simulink model "Sistema3"  (R2026b)
settings: Solver=ode15s  StopTime=10  MaxStep=1E-2
libraries: slpidlib x1
settings Model: LastModifiedBy=Marcos Ancelmo
settings DataIOCC: DSMLogging=off  ReturnWorkspaceOutputs=off  SaveFormat=Array  SaveOutput=off  SignalLogging=off  TimeSaveName=t
settings DebuggingCC: AlgebraicLoopMsg=none  ArtificialAlgebraicLoopMsg=none  MaxConsecutiveZCsMsg=none

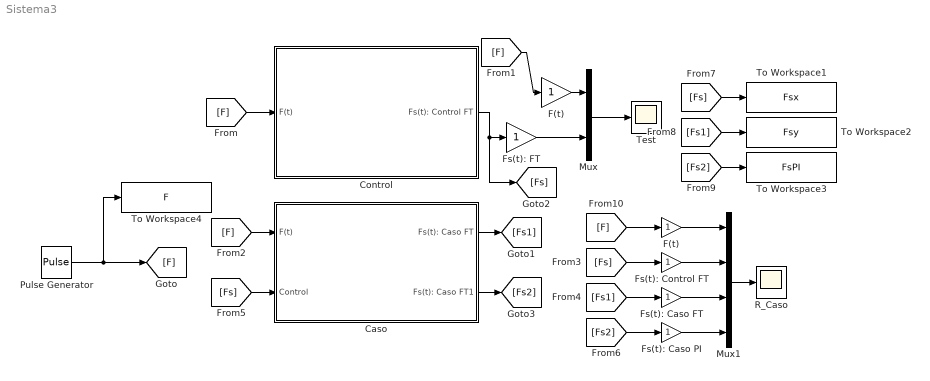
== system Sistema3 ==
  " F(t)" : Gain
  " Fs(t): Caso FT" : Gain
  " Fs(t): Caso PI" : Gain
  " Fs(t): Control FT" : Gain
  Caso : Subsystem
  Control : Subsystem
  F(t) : Gain
  Fs(t): FT : Gain
  Mux : Mux  Inputs=2
  Mux1 : Mux
  Pulse Generator : DiscretePulseGenerator  PulseType=Time based  Period=10  PulseWidth=10  PhaseDelay=1
  R_Caso : Scope
      settings: ActiveDisplayYMinimum=-0.12564340388071826  ActiveDisplayYMaximum=1.1250714893200797
  Test : Scope
      settings: ActiveDisplayYMinimum=-0.12500093230348591  ActiveDisplayYMaximum=1.1250001035892763
  To Workspace1 : ToWorkspace  VariableName=Fsx  SampleTime=-1
  To Workspace2 : ToWorkspace  VariableName=Fsy  SampleTime=-1
  To Workspace3 : ToWorkspace  VariableName=FsPI  SampleTime=-1
  To Workspace4 : ToWorkspace  VariableName=F  SampleTime=-1
  wires:
  Mux/1 -> Test/1
  [F] -> Control/1(F(t))
  Fs(t): FT/1 -> Mux/2
  Control/1(Fs(t): Control FT) -> [Fs], Fs(t): FT/1
  [F] -> Caso/1(F(t))
  Caso/1(Fs(t): Caso FT) -> [Fs1]
  Mux1/1 -> R_Caso/1
  [Fs] -> " Fs(t): Control FT"/1
  [Fs1] -> " Fs(t): Caso FT"/1
  Pulse Generator/1 -> To Workspace4/1, [F]
  [Fs] -> Caso/2(Control)
  Caso/2(Fs(t): Caso FT1) -> [Fs2]
  [Fs2] -> " Fs(t): Caso PI"/1
  [Fs] -> To Workspace1/1
  [Fs1] -> To Workspace2/1
  [Fs2] -> To Workspace3/1
  F(t)/1 -> Mux/1
  [F] -> F(t)/1
  [F] -> " F(t)"/1
  " Fs(t): Control FT"/1 -> Mux1/2
  " F(t)"/1 -> Mux1/1
  " Fs(t): Caso FT"/1 -> Mux1/3
  " Fs(t): Caso PI"/1 -> Mux1/4

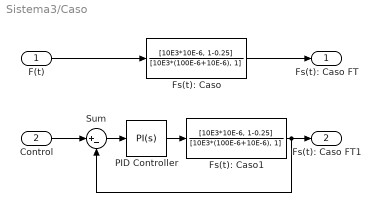
== system Sistema3/Caso ==
  F(t) : Inport
  Control : Inport  Port=2
  Fs(t): Caso : TransferFcn  Numerator=[10E3*10E-6, 1-0.25]  Denominator=[10E3*(100E-6+10E-6), 1]
  Fs(t): Caso1 : TransferFcn  Numerator=[10E3*10E-6, 1-0.25]  Denominator=[10E3*(100E-6+10E-6), 1]
  PID Controller : slpidlib/PID Controller  Controller=PI  Form=Parallel  TimeDomain=Continuous-time  UseExternalTs=off  SampleTime=-1  IntegratorMethod=Forward Euler  FilterMethod=Forward Euler  ControllerParametersSource=internal  P=0.0215035428234307  I=42202.0255640197  UseKiTs=off  D=0  UseExternalDerivativeSource=off  N=100  UseFilter=on  TunerSelectOption=Transfer Function Based (PID Tuner App)  InitialConditionSource=internal  InitialConditionForIntegrator=0  InitialConditionForFilter=0  DifferentiatorICPrevScaledInput=0  ExternalReset=none  TrackingMode=off  Kt=1  LimitOutput=off  SatLimitsSource=internal  UpperSaturationLimit=inf  LowerSaturationLimit=-inf  LinearizeAsGain=on  AntiWindupMode=none  Kb=1  LimitIntegrator=off  UpperIntegratorSaturationLimit=inf  LowerIntegratorSaturationLimit=-inf  POutMin=[]  POutMax=[]  IOutMin=[]  IOutMax=[]  DOutMin=[]  DOutMax=[]  NOutMin=[]  NOutMax=[]  SumOutMin=[]  SumOutMax=[]  SaturationOutMin=[]  SaturationOutMax=[]  PParamMin=[]  PParamMax=[]  IParamMin=[]  IParamMax=[]  DParamMin=[]  DParamMax=[]  NParamMin=[]  NParamMax=[]  KbParamMin=[]  KbParamMax=[]  KtParamMin=[]  KtParamMax=[]  KbOutMin=[]  KbOutMax=[]  KtOutMin=[]  KtOutMax=[]  IntegratorOutMin=[]  IntegratorOutMax=[]  FilterOutMin=[]  FilterOutMax=[]  SumI1OutMin=[]  SumI1OutMax=[]  SumI2OutMin=[]  SumI2OutMax=[]  SumI3OutMin=[]  SumI3OutMax=[]  SumI4OutMin=[]  SumI4OutMax=[]  SumDOutMin=[]  SumDOutMax=[]  DifferentiatorOutMin=[]  DifferentiatorOutMax=[]  FilterDiffOutCoefMin=[]  FilterDiffOutCoefMax=[]  ReciprocalOutMin=[]  ReciprocalOutMax=[]  SumDenOutMin=[]  SumDenOutMax=[]  SumNumOutMin=[]  SumNumOutMax=[]  DivideOutMin=[]  DivideOutMax=[]  UdiffTsProdOutMin=[]  UdiffTsProdOutMax=[]  NTsProdOutMin=[]  NTsProdOutMax=[]  UintegralTsProdOutMin=[]  UintegralTsProdOutMax=[]  UngainTsProdOutMin=[]  UngainTsProdOutMax=[]  ClampingZeroOutDataTypeStr=Inherit: Inherit via back propagation  ClampingZeroOutMin=[]  ClampingZeroOutMax=[]  FilterDenConstantOutDataTypeStr=Inherit: Inherit via back propagation  FilterDenConstantOutMin=[]  FilterDenConstantOutMax=[]  PCopyOutDataTypeStr=Inherit: Inherit via back propagation  PCopyOutMin=[]  PCopyOutMax=[]  NCopyOutDataTypeStr=Inherit: Inherit via back propagation  NCopyOutMin=[]  NCopyOutMax=[]  IntegratorContinuousStateAttributes=''  IntegratorStateMustResolveToSignalObject=off  IntegratorRTWStateStorageClass=Auto  FilterContinuousStateAttributes=''  FilterStateMustResolveToSignalObject=off  FilterRTWStateStorageClass=Auto  ParallelPVariant=InternalParameters  IdealPVariant=Disabled  IVariant=InternalParameters  DVariant=Disabled  IntegratorVariant=Continuous  SatVariant=Disabled  AWVariant=Passthrough  PCopyVariant=Disabled  TRVariant=Disabled  FdbkBlocksVariant=Forward  IdealPFdbkVariant=Disabled  SatFdbkVariant=Disabled  DerivativeFilterVariant=Disabled  NVariant=Disabled  NCopyVariant=Disabled_SignalSpec  FilterICVariant=Disabled  IntegratorICVariant=InternalICs  ExternalResetVariant=Disabled  TRSumVariant=Passthrough  SumFdbkVariant=Disabled  SumVariant=Sum_PI  TsampFilterVariant=InternalTs  TsampNgainVariant=Passthrough  TsampIntegralVariant=Disabled_SignalSpec  ExternalSaturationOutDataTypeStr=Inherit: Same as second input  DerivativeSourceVariant=Disabled  PreIntVariant=InternalPreInt
  Sum : Sum  Inputs=|+-
  Fs(t): Caso FT : Outport
  Fs(t): Caso FT1 : Outport  Port=2
  wires:
  F(t)/1 -> Fs(t): Caso/1
  Fs(t): Caso/1 -> Fs(t): Caso FT/1
  PID Controller/1 -> Fs(t): Caso1/1
  Sum/1 -> PID Controller/1
  Fs(t): Caso1/1 -> Fs(t): Caso FT1/1, Sum/2
  Control/1 -> Sum/1

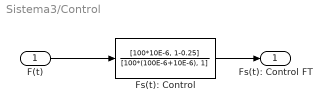
== system Sistema3/Control ==
  F(t) : Inport
  Fs(t): Control : TransferFcn  Numerator=[100*10E-6, 1-0.25]  Denominator=[100*(100E-6+10E-6), 1]
  Fs(t): Control FT : Outport
  wires:
  F(t)/1 -> Fs(t): Control/1
  Fs(t): Control/1 -> Fs(t): Control FT/1
